simulink model "Low_speed_sim"  (R2016a)
settings: Solver=VariableStepAuto  StartTime=0.0  StopTime=100  RelTol=1e-3
values from neighbouring files (symbols this model uses):
  Kp1 = cp1*wL    (= 1.68)    [Low_speed.m]
libraries: simulink x1
settings Model: Creator=DELL  LastModifiedBy=DELL

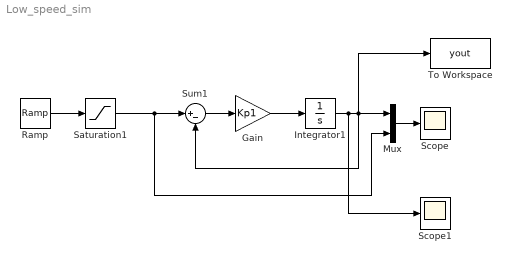
== system Low_speed_sim ==
  Gain : Gain  Gain=Kp1
  Integrator1 : Integrator
  Mux : Mux  Inputs=2
  Ramp : simulink/Sources/Ramp  slope=1  start=0  X0=0
  Saturation1 : Saturate  UpperLimit=10  LowerLimit=0
  Scope : Scope
  Scope1 : Scope
  Sum1 : Sum  Inputs=|+-
  To Workspace : ToWorkspace  VariableName=yout  SaveFormat=Timeseries  SampleTime=-1
  wires:
  Ramp/1 -> Saturation1/1
  Saturation1/1 -> Mux/2, Sum1/1
  Mux/1 -> Scope/1
  Sum1/1 -> Gain/1
  Gain/1 -> Integrator1/1
  Integrator1/1 -> Scope1/1, To Workspace/1, Sum1/2, Mux/1
